simulink model "MRAC_T2"  (R2023b)
settings: Solver=VariableStepAuto  StartTime=0.0  StopTime=60  MaxStep=0.001  RelTol=1e-3
values from neighbouring files (symbols this model uses):
  A = [ ... (first row only)    [MRAC_T2.m]    (also in taller_MRAC_directo.m = [-0.0175, 0.173,   -9.77,     -5.63)
  B = [-0.428; 4.91; 0; 4.22]    [MRAC_T2.m]    (also in taller_MRAC_directo.m)
  Cm = eye(4,4)    [MRAC_T2.m]
  Dm = zeros(4,1)    [MRAC_T2.m]
libraries: slctrl_adaptive x1, simulink x1
settings Model: Creator=sslan  LastModifiedBy=sslan

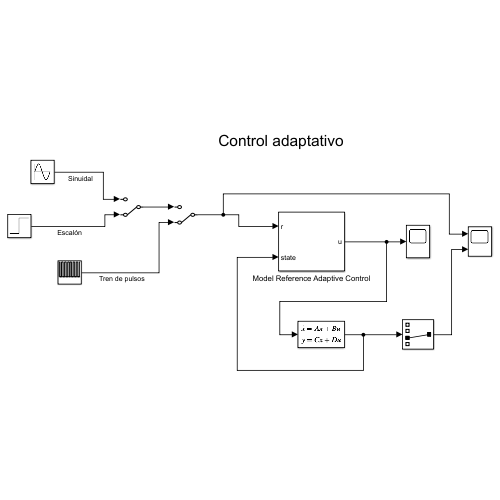
[thumbnail: Simulink's stored preview of the top-level diagram]
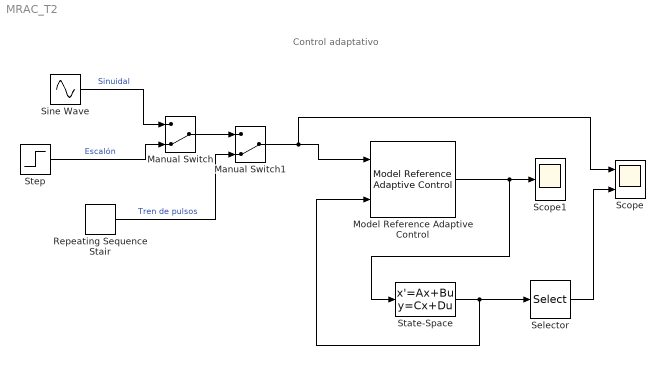
== system MRAC_T2 ==
  note: Control adaptativo
  Manual Switch : ManualSwitch  CurrentSetting=0
  Manual Switch1 : ManualSwitch  CurrentSetting=0
  Model Reference Adaptive Control : slctrl_adaptive/Model Reference Adaptive Control  selectType=Direct  A=A  B=B  Ahat=0  ALrEnable=on  gamma_a=1  ALrEnableMod=on  Bhat=1  BLrEnable=on  gamma_b=1  BLrEnableMod=on  externalKtauEnable=off  k_tau=-1  estParamOutput=off  Am=Am  Bm=Bm  kx=0  FBLrEnable=on  gamma_kx=100  FBLrEnableMod=on  kr=0  FFLrEnable=on  gamma_kr=100  FFLrEnableMod=on  AdaptEnable=on  gamma=1  WLrEnableMod=on  Q=100  FeatureTypeOptions=State  shlHiddenLayerSize=10  gamma_V=0.1  nCen=20  cSpanMin=-1  cSpanMax=1  cSig=5  adaptiveCntrlOutport=off  modChoice=None  sigma_val=0.1
      settings: LibrarySourceBlock=slctrlblks/Adaptive Control/Model Reference Adaptive Control
  Repeating Sequence Stair : simulink/Sources/Repeating Sequence Stair  OutValues=[2 0 2 0 2 0 2 0 2 0 2 0 2 0 2].'  tsamp=5  OutMin=[]  OutMax=[]  OutDataTypeStr=double  OutputDataTypeScalingMode=double  OutDataType=fixdt(0,8)  ConRadixGroup=Best Precision: Vector-wise  OutScaling=2^-12
  Scope : Scope  NumInputPorts=2
  Scope1 : Scope
  Selector : Selector  InputPortWidth=4  IndexOptions=Index vector (dialog)  Indices=[3]  OutputSizes=1
  Sine Wave : Sin  SampleTime=0
  State-Space : StateSpace  A=A  B=B  C=Cm  D=Dm  InitialCondition=0
  Step : Step  SampleTime=0
  wires:
  Model Reference Adaptive Control/1 -> State-Space/1, Scope1/1
  State-Space/1 -> Model Reference Adaptive Control/2, Selector/1
  Selector/1 -> Scope/2
  Sine Wave/1 -> Manual Switch/1  "Sinuidal"
  Step/1 -> Manual Switch/2  "Escalón"
  Repeating Sequence Stair/1 -> Manual Switch1/2  "Tren de pulsos"
  Manual Switch/1 -> Manual Switch1/1
  Manual Switch1/1 -> Scope/1, Model Reference Adaptive Control/1
